simulink model "FlightSim_6DOF"  (R2026b)
settings: Solver=VariableStepAuto
values from neighbouring files (symbols this model uses):
  feet_pos_body_m = [ -1.87  -1.87  -1.87  -1.87 ... (first row only)    [FS_6DOF_config.m]
  g = 9.81    [FS_6DOF_config.m]    (also in hornet_sim_1D_init.m)
  PID_KD_pitch = 0.0    (= 0)    [FS_6DOF_config.m]
  PID_KD_yaw = 0.0    (= 0)    [FS_6DOF_config.m]
  PID_KI_pitch = 0.0    (= 0)    [FS_6DOF_config.m]
  PID_KI_yaw = 0.0    (= 0)    [FS_6DOF_config.m]
  PID_KP_pitch = 0.0    (= 0)    [FS_6DOF_config.m]
  PID_KP_yaw = 0.0    (= 0)    [FS_6DOF_config.m]
  PIDX_KD_pos = 0.0    (= 0)    [FS_6DOF_config.m]
  PIDX_KI_pos = 0.0    (= 0)    [FS_6DOF_config.m]
  PIDX_KP_pos = 0.0    (= 0)    [FS_6DOF_config.m]
  PIDY_KD_pos = 0.0    (= 0)    [FS_6DOF_config.m]
  PIDY_KI_pos = 0.0    (= 0)    [FS_6DOF_config.m]
  PIDY_KP_pos = 0.0    (= 0)    [FS_6DOF_config.m]
  PIDZ_KD_pos = 0.0    (= 0)    [FS_6DOF_config.m]
  PIDZ_KD_vel = 0.0    (= 0)    [FS_6DOF_config.m]
  PIDZ_KI_pos = 0.0    (= 0)    [FS_6DOF_config.m]
  PIDZ_KI_vel = 0.0    (= 0)    [FS_6DOF_config.m]
  PIDZ_KP_pos = 0.0    (= 0)    [FS_6DOF_config.m]
  PIDZ_KP_vel = 0.0    (= 0)    [FS_6DOF_config.m]
  pitch0 = 0.0    (= 0)    [FS_6DOF_config.m]
  Position_Target_inertial = [x_targ; y_targ;z_targ]    [FS_6DOF_config.m]
  roll0 = 0.0    (= 0)    [FS_6DOF_config.m]
  vx0 = 0    [FS_6DOF_config.m]    (also in hornet_sim_1D_init.m)
  vy0 = 0    [FS_6DOF_config.m]
  vz0 = 0    [FS_6DOF_config.m]
  x0 = 0    [FS_6DOF_config.m]    (also in hornet_sim_1D_init.m = 1)
  x_hat_body = [1;0;0]    [FS_6DOF_config.m]
  y0 = 0    [FS_6DOF_config.m]
  yaw0 = 0.0    (= 0)    [FS_6DOF_config.m]
  z0 = 0    [FS_6DOF_config.m]
undefined symbols (not defined in the file or in its folder): DiscIntNeverNeededParam, Lidar_1, Lidar_2, veh, VN300Config
libraries: aerolibutil x8, slpidlib x5, sharedutil x2, matrix_library x1
settings Model: Creator=11and  LastModifiedBy=jet
settings RTWCC: GenCodeOnly=on
settings SimscapeCC: SimscapeLogType=all  SimscapeNominalValues="[{\"value\":\"1\",\"unit\":\"A\"},{\"value\":\"1\",\"unit\":\"bar\"},{\"value\":\"1\",\"unit\":\"cm^2\"},{\"value\":\"1\",\"unit\":\"cm^3/s\"},{\"value\":\"1\",\"unit\":\"kJ/kg\"},{\"value\":\"1\",\"unit\":\"kW\"},{\"value\":\"1\",\"unit\":\"l\"},{\"value\":\"1\",\"unit\":\"N\"},{\"value\":\"1\",\"unit\":\"N*m\"},{\"value\":\"1\",\"unit\":\"V\"},{\"value\":\"0.001\",\"unit\":\"Wb\"}]"  SimscapeUseEnergyAccounting=off

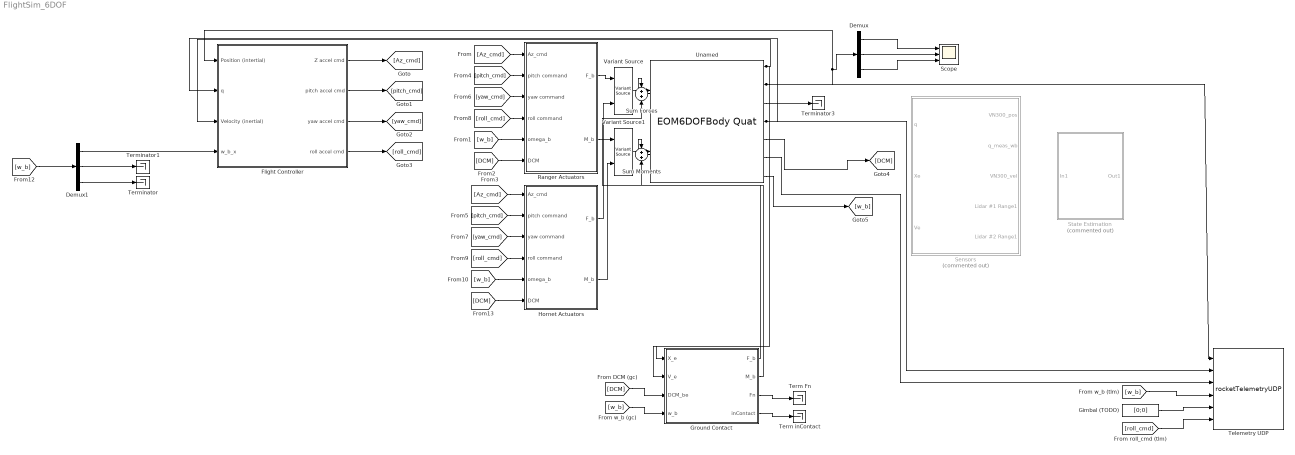
== system FlightSim_6DOF ==
  Demux : Demux  Outputs=3
  Demux1 : Demux  Outputs=3
  Flight Controller : Subsystem
  Gimbal (TODO) : Constant  Value=[0;0]
  Ground Contact : MATLAB Function  TreatAsAtomicUnit=on
  Hornet Actuators : Subsystem
  Ranger Actuators : Subsystem
  Scope : Scope  NumInputPorts=3
      settings: ActiveDisplayYMinimum=-236.81123475820692  ActiveDisplayYMaximum=587.41234905749616
  Sensors : Subsystem  Commented=on
  State Estimation : Subsystem  Commented=on
  Sum Forces : Sum
  Sum Moments : Sum
  Telemetry UDP : M-S-Function  FunctionName=rocketTelemetryUDP
      mask Display:
      | port_label('input', 1, 'position_e');
      | port_label('input', 2, 'quaternion_eb');
      | port_label('input', 3, 'velocity_b');
      | port_label('input', 4, 'omega_b');
      | port_label('input', 5, 'gimbal');
      | port_label('input', 6, 'rcs');
  Term Fn : Terminator
  Term inContact : Terminator
  Terminator : Terminator
  Terminator1 : Terminator
  Terminator3 : Terminator
  Unamed : EOM6DOFBodyQuat  xme_0=[x0 y0 z0]  Vm_0=[vx0 vy0 vz0]  eul_0=[roll0 pitch0 yaw0]  mass_0=veh.m  inertia=veh.I
  Variant Source : VariantSource  VariantControls={VEHICLE == 1, VEHICLE == 2}
  Variant Source1 : VariantSource  VariantControls={VEHICLE == 1, VEHICLE == 2}
  wires:
  Unamed/2 -> Flight Controller/1(Position (intertial)), Demux/1, Telemetry UDP/1, Ground Contact/1(X_e)
  Demux/1 -> Scope/1
  Demux/2 -> Scope/2
  Demux/3 -> Scope/3
  Unamed/4 -> Flight Controller/2(q), Telemetry UDP/2
  Unamed/7 -> [w_b]
  Unamed/1 -> Flight Controller/3(Velocity (inertial)), Ground Contact/2(V_e)
  Demux1/3 -> Terminator/1
  Demux1/2 -> Terminator1/1
  Demux1/1 -> Flight Controller/4(w_b_x)
  Unamed/3 -> Terminator3/1
  Unamed/5 -> [DCM]
  [w_b] -> Demux1/1
  Flight Controller/1(Z accel cmd) -> [Az_cmd]
  Flight Controller/2(pitch accel cmd) -> [pitch_cmd]
  [w_b] -> Hornet Actuators/5(omega_b)
  Ranger Actuators/1(F_b) -> Variant Source/1
  Flight Controller/3(yaw accel cmd) -> [yaw_cmd]
  Flight Controller/4(roll accel cmd) -> [roll_cmd]
  [DCM] -> Hornet Actuators/6(DCM)
  Hornet Actuators/1(F_b) -> Variant Source/2
  Ranger Actuators/2(M_b) -> Variant Source1/1
  Hornet Actuators/2(M_b) -> Variant Source1/2
  [w_b] -> Ranger Actuators/5(omega_b)
  [DCM] -> Ranger Actuators/6(DCM)
  [Az_cmd] -> Ranger Actuators/1(Az_cmd)
  [Az_cmd] -> Hornet Actuators/1(Az_cmd)
  [pitch_cmd] -> Ranger Actuators/2(pitch command)
  [pitch_cmd] -> Hornet Actuators/2(pitch command)
  [yaw_cmd] -> Ranger Actuators/3(yaw command)
  [yaw_cmd] -> Hornet Actuators/3(yaw command)
  [roll_cmd] -> Ranger Actuators/4(roll command)
  [roll_cmd] -> Hornet Actuators/4(roll command)
  Unamed/6 -> Telemetry UDP/3
  [w_b] -> Telemetry UDP/4
  Gimbal (TODO)/1 -> Telemetry UDP/5
  [roll_cmd] -> Telemetry UDP/6
  [DCM] -> Ground Contact/3(DCM_be)
  [w_b] -> Ground Contact/4(w_b)
  Ground Contact/3(Fn) -> Term Fn/1
  Ground Contact/4(inContact) -> Term inContact/1
  Variant Source/1 -> Sum Forces/1
  Ground Contact/1(F_b) -> Sum Forces/2
  Sum Forces/1 -> Unamed/1
  Variant Source1/1 -> Sum Moments/1
  Ground Contact/2(M_b) -> Sum Moments/2
  Sum Moments/1 -> Unamed/2

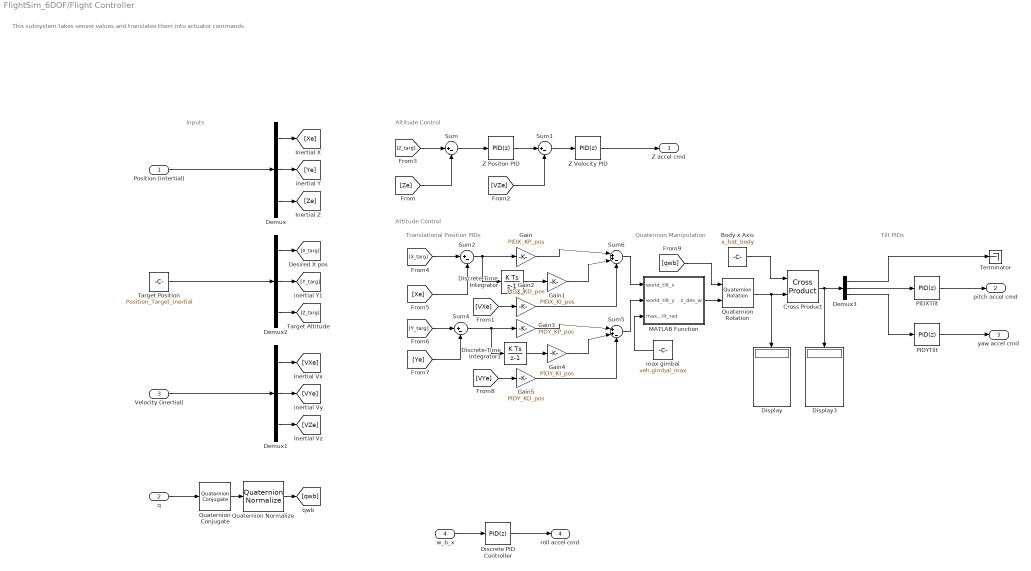
== system FlightSim_6DOF/Flight Controller ==
  note: This subsystem takes sensor values and translates them into actuator commands
  note: Tilt PIDs
  note: Quaternion Manipulation
  note: Translational Position PIDs
  note: Inputs
  note: Attitude Control
  note: Altitude Control
  Position (intertial) : Inport
  q : Inport  Port=2
  Velocity (inertial) : Inport  Port=3
  w_b_x : Inport  Port=4
  Body x Axis : Constant  Value=x_hat_body
  Cross Product : matrix_library/Cross Product
  Demux{,1..3} (4 alike) : Demux  Outputs=3
  Discrete PID Controller : slpidlib/PID Controller  Controller=PID  Form=Parallel  TimeDomain=Discrete-time  UseExternalTs=off  SampleTime=-1  IntegratorMethod=Forward Euler  FilterMethod=Forward Euler  ControllerParametersSource=internal  P=1  I=1  UseKiTs=off  D=0  UseExternalDerivativeSource=off  N=100  UseFilter=on  TunerSelectOption=Transfer Function Based (PID Tuner App)  InitialConditionSource=internal  InitialConditionForIntegrator=0  InitialConditionForFilter=0  DifferentiatorICPrevScaledInput=0  ExternalReset=none  TrackingMode=off  Kt=1  LimitOutput=off  SatLimitsSource=internal  UpperSaturationLimit=inf  LowerSaturationLimit=-inf  LinearizeAsGain=off  AntiWindupMode=none  Kb=1  LimitIntegrator=off  UpperIntegratorSaturationLimit=inf  LowerIntegratorSaturationLimit=-inf  POutMin=[]  POutMax=[]  IOutMin=[]  IOutMax=[]  DOutMin=[]  DOutMax=[]  NOutMin=[]  NOutMax=[]  SumOutMin=[]  SumOutMax=[]  SaturationOutMin=[]  SaturationOutMax=[]  PParamMin=[]  PParamMax=[]  IParamMin=[]  IParamMax=[]  DParamMin=[]  DParamMax=[]  NParamMin=[]  NParamMax=[]  KbParamMin=[]  KbParamMax=[]  KtParamMin=[]  KtParamMax=[]  KbOutMin=[]  KbOutMax=[]  KtOutMin=[]  KtOutMax=[]  IntegratorOutMin=[]  IntegratorOutMax=[]  FilterOutMin=[]  FilterOutMax=[]  SumI1OutMin=[]  SumI1OutMax=[]  SumI2OutMin=[]  SumI2OutMax=[]  SumI3OutMin=[]  SumI3OutMax=[]  SumI4OutMin=[]  SumI4OutMax=[]  SumDOutMin=[]  SumDOutMax=[]  DifferentiatorOutMin=[]  DifferentiatorOutMax=[]  FilterDiffOutCoefMin=[]  FilterDiffOutCoefMax=[]  ReciprocalOutMin=[]  ReciprocalOutMax=[]  SumDenOutMin=[]  SumDenOutMax=[]  SumNumOutMin=[]  SumNumOutMax=[]  DivideOutMin=[]  DivideOutMax=[]  UdiffTsProdOutMin=[]  UdiffTsProdOutMax=[]  NTsProdOutMin=[]  NTsProdOutMax=[]  UintegralTsProdOutMin=[]  UintegralTsProdOutMax=[]  UngainTsProdOutMin=[]  UngainTsProdOutMax=[]  ClampingZeroOutDataTypeStr=Inherit: Inherit via back propagation  ClampingZeroOutMin=[]  ClampingZeroOutMax=[]  FilterDenConstantOutDataTypeStr=Inherit: Inherit via back propagation  FilterDenConstantOutMin=[]  FilterDenConstantOutMax=[]  PCopyOutDataTypeStr=Inherit: Inherit via back propagation  PCopyOutMin=[]  PCopyOutMax=[]  NCopyOutDataTypeStr=Inherit: Inherit via back propagation  NCopyOutMin=[]  NCopyOutMax=[]  IntegratorContinuousStateAttributes=''  IntegratorStateMustResolveToSignalObject=off  IntegratorRTWStateStorageClass=Auto  FilterContinuousStateAttributes=''  FilterStateMustResolveToSignalObject=off  FilterRTWStateStorageClass=Auto  ParallelPVariant=InternalParameters  IdealPVariant=Disabled  IVariant=InternalParameters  DVariant=InternalParameters  IntegratorVariant=Discrete  SatVariant=Disabled  AWVariant=Passthrough  PCopyVariant=Disabled  TRVariant=Disabled  FdbkBlocksVariant=Forward  IdealPFdbkVariant=Disabled  SatFdbkVariant=Disabled  DerivativeFilterVariant=ForwardEulerFilter  NVariant=InternalParameters  NCopyVariant=Disabled  FilterICVariant=InternalICsFilter  IntegratorICVariant=InternalICs  ExternalResetVariant=Disabled  TRSumVariant=Passthrough  SumFdbkVariant=Disabled  SumVariant=Sum_PID  TsampFilterVariant=InternalTs  TsampNgainVariant=Passthrough  TsampIntegralVariant=Disabled_SignalSpec  ExternalSaturationOutDataTypeStr=Inherit: Same as second input  DerivativeSourceVariant=ErrorSignal  PreIntVariant=InternalPreInt
      settings: LibrarySourceBlock=simulink/Discrete/Discrete PID Controller
  Discrete-Time Integrator : DiscreteIntegrator  SampleTime=-1  ICPrevOutput=DiscIntNeverNeededParam  ICPrevScaledInput=DiscIntNeverNeededParam
  Discrete-Time Integrator1 : DiscreteIntegrator  SampleTime=-1  ICPrevOutput=DiscIntNeverNeededParam  ICPrevScaledInput=DiscIntNeverNeededParam
  Display : Display
  Display3 : Display
  Gain : Gain  Gain=PIDX_KP_pos
  Gain1 : Gain  Gain=PIDX_KI_pos
  Gain2 : Gain  Gain=PIDX_KD_pos
  Gain3 : Gain  Gain=PIDY_KP_pos
  Gain4 : Gain  Gain=PIDY_KI_pos
  Gain5 : Gain  Gain=PIDY_KD_pos
  MATLAB Function : MATLAB Function  TreatAsAtomicUnit=on
  PIDXTilt : slpidlib/PID Controller  Controller=PID  Form=Parallel  TimeDomain=Discrete-time  UseExternalTs=off  SampleTime=-1  IntegratorMethod=Forward Euler  FilterMethod=Forward Euler  ControllerParametersSource=internal  P=PID_KP_pitch  I=PID_KI_pitch  UseKiTs=off  D=PID_KD_pitch  UseExternalDerivativeSource=off  N=100  UseFilter=on  TunerSelectOption=Transfer Function Based (PID Tuner App)  InitialConditionSource=internal  InitialConditionForIntegrator=0  InitialConditionForFilter=0  DifferentiatorICPrevScaledInput=0  ExternalReset=none  TrackingMode=off  Kt=1  LimitOutput=off  SatLimitsSource=internal  UpperSaturationLimit=inf  LowerSaturationLimit=-inf  LinearizeAsGain=off  AntiWindupMode=none  Kb=1  LimitIntegrator=off  UpperIntegratorSaturationLimit=inf  LowerIntegratorSaturationLimit=-inf  POutMin=[]  POutMax=[]  IOutMin=[]  IOutMax=[]  DOutMin=[]  DOutMax=[]  NOutMin=[]  NOutMax=[]  SumOutMin=[]  SumOutMax=[]  SaturationOutMin=[]  SaturationOutMax=[]  PParamMin=[]  PParamMax=[]  IParamMin=[]  IParamMax=[]  DParamMin=[]  DParamMax=[]  NParamMin=[]  NParamMax=[]  KbParamMin=[]  KbParamMax=[]  KtParamMin=[]  KtParamMax=[]  KbOutMin=[]  KbOutMax=[]  KtOutMin=[]  KtOutMax=[]  IntegratorOutMin=[]  IntegratorOutMax=[]  FilterOutMin=[]  FilterOutMax=[]  SumI1OutMin=[]  SumI1OutMax=[]  SumI2OutMin=[]  SumI2OutMax=[]  SumI3OutMin=[]  SumI3OutMax=[]  SumI4OutMin=[]  SumI4OutMax=[]  SumDOutMin=[]  SumDOutMax=[]  DifferentiatorOutMin=[]  DifferentiatorOutMax=[]  FilterDiffOutCoefMin=[]  FilterDiffOutCoefMax=[]  ReciprocalOutMin=[]  ReciprocalOutMax=[]  SumDenOutMin=[]  SumDenOutMax=[]  SumNumOutMin=[]  SumNumOutMax=[]  DivideOutMin=[]  DivideOutMax=[]  UdiffTsProdOutMin=[]  UdiffTsProdOutMax=[]  NTsProdOutMin=[]  NTsProdOutMax=[]  UintegralTsProdOutMin=[]  UintegralTsProdOutMax=[]  UngainTsProdOutMin=[]  UngainTsProdOutMax=[]  ClampingZeroOutDataTypeStr=Inherit: Inherit via back propagation  ClampingZeroOutMin=[]  ClampingZeroOutMax=[]  FilterDenConstantOutDataTypeStr=Inherit: Inherit via back propagation  FilterDenConstantOutMin=[]  FilterDenConstantOutMax=[]  PCopyOutDataTypeStr=Inherit: Inherit via back propagation  PCopyOutMin=[]  PCopyOutMax=[]  NCopyOutDataTypeStr=Inherit: Inherit via back propagation  NCopyOutMin=[]  NCopyOutMax=[]  IntegratorContinuousStateAttributes=''  IntegratorStateMustResolveToSignalObject=off  IntegratorRTWStateStorageClass=Auto  FilterContinuousStateAttributes=''  FilterStateMustResolveToSignalObject=off  FilterRTWStateStorageClass=Auto  ParallelPVariant=InternalParameters  IdealPVariant=Disabled  IVariant=InternalParameters  DVariant=InternalParameters  IntegratorVariant=Discrete  SatVariant=Disabled  AWVariant=Passthrough  PCopyVariant=Disabled  TRVariant=Disabled  FdbkBlocksVariant=Forward  IdealPFdbkVariant=Disabled  SatFdbkVariant=Disabled  DerivativeFilterVariant=ForwardEulerFilter  NVariant=InternalParameters  NCopyVariant=Disabled  FilterICVariant=InternalICsFilter  IntegratorICVariant=InternalICs  ExternalResetVariant=Disabled  TRSumVariant=Passthrough  SumFdbkVariant=Disabled  SumVariant=Sum_PID  TsampFilterVariant=InternalTs  TsampNgainVariant=Passthrough  TsampIntegralVariant=Disabled_SignalSpec  ExternalSaturationOutDataTypeStr=Inherit: Same as second input  DerivativeSourceVariant=ErrorSignal  PreIntVariant=InternalPreInt
      settings: LibrarySourceBlock=simulink/Discrete/Discrete PID Controller
  PIDYTilt : slpidlib/PID Controller  Controller=PID  Form=Parallel  TimeDomain=Discrete-time  UseExternalTs=off  SampleTime=-1  IntegratorMethod=Forward Euler  FilterMethod=Forward Euler  ControllerParametersSource=internal  P=PID_KP_yaw  I=PID_KI_yaw  UseKiTs=off  D=PID_KD_yaw  UseExternalDerivativeSource=off  N=100  UseFilter=on  TunerSelectOption=Transfer Function Based (PID Tuner App)  InitialConditionSource=internal  InitialConditionForIntegrator=0  InitialConditionForFilter=0  DifferentiatorICPrevScaledInput=0  ExternalReset=none  TrackingMode=off  Kt=1  LimitOutput=off  SatLimitsSource=internal  UpperSaturationLimit=inf  LowerSaturationLimit=-inf  LinearizeAsGain=off  AntiWindupMode=none  Kb=1  LimitIntegrator=off  UpperIntegratorSaturationLimit=inf  LowerIntegratorSaturationLimit=-inf  POutMin=[]  POutMax=[]  IOutMin=[]  IOutMax=[]  DOutMin=[]  DOutMax=[]  NOutMin=[]  NOutMax=[]  SumOutMin=[]  SumOutMax=[]  SaturationOutMin=[]  SaturationOutMax=[]  PParamMin=[]  PParamMax=[]  IParamMin=[]  IParamMax=[]  DParamMin=[]  DParamMax=[]  NParamMin=[]  NParamMax=[]  KbParamMin=[]  KbParamMax=[]  KtParamMin=[]  KtParamMax=[]  KbOutMin=[]  KbOutMax=[]  KtOutMin=[]  KtOutMax=[]  IntegratorOutMin=[]  IntegratorOutMax=[]  FilterOutMin=[]  FilterOutMax=[]  SumI1OutMin=[]  SumI1OutMax=[]  SumI2OutMin=[]  SumI2OutMax=[]  SumI3OutMin=[]  SumI3OutMax=[]  SumI4OutMin=[]  SumI4OutMax=[]  SumDOutMin=[]  SumDOutMax=[]  DifferentiatorOutMin=[]  DifferentiatorOutMax=[]  FilterDiffOutCoefMin=[]  FilterDiffOutCoefMax=[]  ReciprocalOutMin=[]  ReciprocalOutMax=[]  SumDenOutMin=[]  SumDenOutMax=[]  SumNumOutMin=[]  SumNumOutMax=[]  DivideOutMin=[]  DivideOutMax=[]  UdiffTsProdOutMin=[]  UdiffTsProdOutMax=[]  NTsProdOutMin=[]  NTsProdOutMax=[]  UintegralTsProdOutMin=[]  UintegralTsProdOutMax=[]  UngainTsProdOutMin=[]  UngainTsProdOutMax=[]  ClampingZeroOutDataTypeStr=Inherit: Inherit via back propagation  ClampingZeroOutMin=[]  ClampingZeroOutMax=[]  FilterDenConstantOutDataTypeStr=Inherit: Inherit via back propagation  FilterDenConstantOutMin=[]  FilterDenConstantOutMax=[]  PCopyOutDataTypeStr=Inherit: Inherit via back propagation  PCopyOutMin=[]  PCopyOutMax=[]  NCopyOutDataTypeStr=Inherit: Inherit via back propagation  NCopyOutMin=[]  NCopyOutMax=[]  IntegratorContinuousStateAttributes=''  IntegratorStateMustResolveToSignalObject=off  IntegratorRTWStateStorageClass=Auto  FilterContinuousStateAttributes=''  FilterStateMustResolveToSignalObject=off  FilterRTWStateStorageClass=Auto  ParallelPVariant=InternalParameters  IdealPVariant=Disabled  IVariant=InternalParameters  DVariant=InternalParameters  IntegratorVariant=Discrete  SatVariant=Disabled  AWVariant=Passthrough  PCopyVariant=Disabled  TRVariant=Disabled  FdbkBlocksVariant=Forward  IdealPFdbkVariant=Disabled  SatFdbkVariant=Disabled  DerivativeFilterVariant=ForwardEulerFilter  NVariant=InternalParameters  NCopyVariant=Disabled  FilterICVariant=InternalICsFilter  IntegratorICVariant=InternalICs  ExternalResetVariant=Disabled  TRSumVariant=Passthrough  SumFdbkVariant=Disabled  SumVariant=Sum_PID  TsampFilterVariant=InternalTs  TsampNgainVariant=Passthrough  TsampIntegralVariant=Disabled_SignalSpec  ExternalSaturationOutDataTypeStr=Inherit: Same as second input  DerivativeSourceVariant=ErrorSignal  PreIntVariant=InternalPreInt
      settings: LibrarySourceBlock=simulink/Discrete/Discrete PID Controller
  Quaternion Conjugate : aerolibutil/Quaternion Conjugate
  Quaternion Normalize : sharedutil/Quaternion Normalize  aMode=aMode
  Quaternion Rotation : aerolibutil/Quaternion Rotation
  Sum{,1..2,4} (4 alike) : Sum  Inputs=|+-
  Sum5 : Sum  Inputs=|++-
  Sum6 : Sum  Inputs=|++-
  Target Position : Constant  Value=Position_Target_inertial
  Terminator : Terminator
  Z Positon PID : slpidlib/PID Controller  Controller=PID  Form=Parallel  TimeDomain=Discrete-time  UseExternalTs=off  SampleTime=-1  IntegratorMethod=Forward Euler  FilterMethod=Forward Euler  ControllerParametersSource=internal  P=PIDZ_KP_pos  I=PIDZ_KI_pos  UseKiTs=off  D=PIDZ_KD_pos  UseExternalDerivativeSource=off  N=100  UseFilter=on  TunerSelectOption=Transfer Function Based (PID Tuner App)  InitialConditionSource=internal  InitialConditionForIntegrator=0  InitialConditionForFilter=0  DifferentiatorICPrevScaledInput=0  ExternalReset=none  TrackingMode=off  Kt=1  LimitOutput=off  SatLimitsSource=internal  UpperSaturationLimit=inf  LowerSaturationLimit=-inf  LinearizeAsGain=off  AntiWindupMode=none  Kb=1  LimitIntegrator=off  UpperIntegratorSaturationLimit=inf  LowerIntegratorSaturationLimit=-inf  POutMin=[]  POutMax=[]  IOutMin=[]  IOutMax=[]  DOutMin=[]  DOutMax=[]  NOutMin=[]  NOutMax=[]  SumOutMin=[]  SumOutMax=[]  SaturationOutMin=[]  SaturationOutMax=[]  PParamMin=[]  PParamMax=[]  IParamMin=[]  IParamMax=[]  DParamMin=[]  DParamMax=[]  NParamMin=[]  NParamMax=[]  KbParamMin=[]  KbParamMax=[]  KtParamMin=[]  KtParamMax=[]  KbOutMin=[]  KbOutMax=[]  KtOutMin=[]  KtOutMax=[]  IntegratorOutMin=[]  IntegratorOutMax=[]  FilterOutMin=[]  FilterOutMax=[]  SumI1OutMin=[]  SumI1OutMax=[]  SumI2OutMin=[]  SumI2OutMax=[]  SumI3OutMin=[]  SumI3OutMax=[]  SumI4OutMin=[]  SumI4OutMax=[]  SumDOutMin=[]  SumDOutMax=[]  DifferentiatorOutMin=[]  DifferentiatorOutMax=[]  FilterDiffOutCoefMin=[]  FilterDiffOutCoefMax=[]  ReciprocalOutMin=[]  ReciprocalOutMax=[]  SumDenOutMin=[]  SumDenOutMax=[]  SumNumOutMin=[]  SumNumOutMax=[]  DivideOutMin=[]  DivideOutMax=[]  UdiffTsProdOutMin=[]  UdiffTsProdOutMax=[]  NTsProdOutMin=[]  NTsProdOutMax=[]  UintegralTsProdOutMin=[]  UintegralTsProdOutMax=[]  UngainTsProdOutMin=[]  UngainTsProdOutMax=[]  ClampingZeroOutDataTypeStr=Inherit: Inherit via back propagation  ClampingZeroOutMin=[]  ClampingZeroOutMax=[]  FilterDenConstantOutDataTypeStr=Inherit: Inherit via back propagation  FilterDenConstantOutMin=[]  FilterDenConstantOutMax=[]  PCopyOutDataTypeStr=Inherit: Inherit via back propagation  PCopyOutMin=[]  PCopyOutMax=[]  NCopyOutDataTypeStr=Inherit: Inherit via back propagation  NCopyOutMin=[]  NCopyOutMax=[]  IntegratorContinuousStateAttributes=''  IntegratorStateMustResolveToSignalObject=off  IntegratorRTWStateStorageClass=Auto  FilterContinuousStateAttributes=''  FilterStateMustResolveToSignalObject=off  FilterRTWStateStorageClass=Auto  ParallelPVariant=InternalParameters  IdealPVariant=Disabled  IVariant=InternalParameters  DVariant=InternalParameters  IntegratorVariant=Discrete  SatVariant=Disabled  AWVariant=Passthrough  PCopyVariant=Disabled  TRVariant=Disabled  FdbkBlocksVariant=Forward  IdealPFdbkVariant=Disabled  SatFdbkVariant=Disabled  DerivativeFilterVariant=ForwardEulerFilter  NVariant=InternalParameters  NCopyVariant=Disabled  FilterICVariant=InternalICsFilter  IntegratorICVariant=InternalICs  ExternalResetVariant=Disabled  TRSumVariant=Passthrough  SumFdbkVariant=Disabled  SumVariant=Sum_PID  TsampFilterVariant=InternalTs  TsampNgainVariant=Passthrough  TsampIntegralVariant=Disabled_SignalSpec  ExternalSaturationOutDataTypeStr=Inherit: Same as second input  DerivativeSourceVariant=ErrorSignal  PreIntVariant=InternalPreInt
      settings: LibrarySourceBlock=simulink/Discrete/Discrete PID Controller
  Z Velocity PID : slpidlib/PID Controller  Controller=PID  Form=Parallel  TimeDomain=Discrete-time  UseExternalTs=off  SampleTime=-1  IntegratorMethod=Forward Euler  FilterMethod=Forward Euler  ControllerParametersSource=internal  P=PIDZ_KP_vel  I=PIDZ_KI_vel  UseKiTs=off  D=PIDZ_KD_vel  UseExternalDerivativeSource=off  N=100  UseFilter=on  TunerSelectOption=Transfer Function Based (PID Tuner App)  InitialConditionSource=internal  InitialConditionForIntegrator=0  InitialConditionForFilter=0  DifferentiatorICPrevScaledInput=0  ExternalReset=none  TrackingMode=off  Kt=1  LimitOutput=off  SatLimitsSource=internal  UpperSaturationLimit=inf  LowerSaturationLimit=-inf  LinearizeAsGain=off  AntiWindupMode=none  Kb=1  LimitIntegrator=off  UpperIntegratorSaturationLimit=inf  LowerIntegratorSaturationLimit=-inf  POutMin=[]  POutMax=[]  IOutMin=[]  IOutMax=[]  DOutMin=[]  DOutMax=[]  NOutMin=[]  NOutMax=[]  SumOutMin=[]  SumOutMax=[]  SaturationOutMin=[]  SaturationOutMax=[]  PParamMin=[]  PParamMax=[]  IParamMin=[]  IParamMax=[]  DParamMin=[]  DParamMax=[]  NParamMin=[]  NParamMax=[]  KbParamMin=[]  KbParamMax=[]  KtParamMin=[]  KtParamMax=[]  KbOutMin=[]  KbOutMax=[]  KtOutMin=[]  KtOutMax=[]  IntegratorOutMin=[]  IntegratorOutMax=[]  FilterOutMin=[]  FilterOutMax=[]  SumI1OutMin=[]  SumI1OutMax=[]  SumI2OutMin=[]  SumI2OutMax=[]  SumI3OutMin=[]  SumI3OutMax=[]  SumI4OutMin=[]  SumI4OutMax=[]  SumDOutMin=[]  SumDOutMax=[]  DifferentiatorOutMin=[]  DifferentiatorOutMax=[]  FilterDiffOutCoefMin=[]  FilterDiffOutCoefMax=[]  ReciprocalOutMin=[]  ReciprocalOutMax=[]  SumDenOutMin=[]  SumDenOutMax=[]  SumNumOutMin=[]  SumNumOutMax=[]  DivideOutMin=[]  DivideOutMax=[]  UdiffTsProdOutMin=[]  UdiffTsProdOutMax=[]  NTsProdOutMin=[]  NTsProdOutMax=[]  UintegralTsProdOutMin=[]  UintegralTsProdOutMax=[]  UngainTsProdOutMin=[]  UngainTsProdOutMax=[]  ClampingZeroOutDataTypeStr=Inherit: Inherit via back propagation  ClampingZeroOutMin=[]  ClampingZeroOutMax=[]  FilterDenConstantOutDataTypeStr=Inherit: Inherit via back propagation  FilterDenConstantOutMin=[]  FilterDenConstantOutMax=[]  PCopyOutDataTypeStr=Inherit: Inherit via back propagation  PCopyOutMin=[]  PCopyOutMax=[]  NCopyOutDataTypeStr=Inherit: Inherit via back propagation  NCopyOutMin=[]  NCopyOutMax=[]  IntegratorContinuousStateAttributes=''  IntegratorStateMustResolveToSignalObject=off  IntegratorRTWStateStorageClass=Auto  FilterContinuousStateAttributes=''  FilterStateMustResolveToSignalObject=off  FilterRTWStateStorageClass=Auto  ParallelPVariant=InternalParameters  IdealPVariant=Disabled  IVariant=InternalParameters  DVariant=InternalParameters  IntegratorVariant=Discrete  SatVariant=Disabled  AWVariant=Passthrough  PCopyVariant=Disabled  TRVariant=Disabled  FdbkBlocksVariant=Forward  IdealPFdbkVariant=Disabled  SatFdbkVariant=Disabled  DerivativeFilterVariant=ForwardEulerFilter  NVariant=InternalParameters  NCopyVariant=Disabled  FilterICVariant=InternalICsFilter  IntegratorICVariant=InternalICs  ExternalResetVariant=Disabled  TRSumVariant=Passthrough  SumFdbkVariant=Disabled  SumVariant=Sum_PID  TsampFilterVariant=InternalTs  TsampNgainVariant=Passthrough  TsampIntegralVariant=Disabled_SignalSpec  ExternalSaturationOutDataTypeStr=Inherit: Same as second input  DerivativeSourceVariant=ErrorSignal  PreIntVariant=InternalPreInt
      settings: LibrarySourceBlock=simulink/Discrete/Discrete PID Controller
  max gimbal : Constant  Value=veh.gimbal_max
  Z accel cmd : Outport
  pitch accel cmd : Outport  Port=2
  yaw accel cmd : Outport  Port=3
  roll accel cmd : Outport  Port=4
  wires:
  [Z_targ] -> Sum/1
  Sum/1 -> Z Positon PID/1
  Z Velocity PID/1 -> Z accel cmd/1
  Position (intertial)/1 -> Demux/1
  Demux/1 -> [Xe]
  [Ze] -> Sum/2
  Z Positon PID/1 -> Sum1/1
  Demux1/1 -> [VXe]
  Demux1/2 -> [VYe]
  Demux1/3 -> [VZe]
  [VZe] -> Sum1/2
  Sum1/1 -> Z Velocity PID/1
  Demux2/1 -> [X_targ]
  Demux2/2 -> [Y_targ]
  Demux2/3 -> [Z_targ]
  Sum2/1 -> Discrete-Time Integrator/1, Gain/1
  [X_targ] -> Sum2/1
  [Xe] -> Sum2/2
  [Y_targ] -> Sum4/1
  [Ye] -> Sum4/2
  [VXe] -> Gain2/1
  Gain/1 -> Sum6/1
  Gain2/1 -> Sum6/3
  PIDXTilt/1 -> pitch accel cmd/1
  PIDYTilt/1 -> yaw accel cmd/1
  Gain5/1 -> Sum5/3
  [VYe] -> Gain5/1
  Sum4/1 -> Discrete-Time Integrator1/1, Gain3/1
  Gain3/1 -> Sum5/1
  Sum6/1 -> MATLAB Function/1(world_tilt_x)
  Sum5/1 -> MATLAB Function/2(world_tilt_y)
  MATLAB Function/1(z_des_w) -> Quaternion Rotation/2
  Quaternion Rotation/1 -> Cross Product/2, Display/1
  Body x Axis/1 -> Cross Product/1
  Cross Product/1 -> Demux3/1, Display3/1
  [qwb] -> Quaternion Rotation/1
  Demux3/2 -> PIDXTilt/1
  Demux3/1 -> Terminator/1
  Demux3/3 -> PIDYTilt/1
  Demux/2 -> [Ye]
  Demux/3 -> [Ze]
  Target Position/1 -> Demux2/1
  Quaternion Conjugate/1 -> Quaternion Normalize/1
  q/1 -> Quaternion Conjugate/1
  Quaternion Normalize/1 -> [qwb]
  max gimbal/1 -> MATLAB Function/3(max_tilt_rad)
  Discrete-Time Integrator1/1 -> Gain4/1
  Gain4/1 -> Sum5/2
  Discrete-Time Integrator/1 -> Gain1/1
  Gain1/1 -> Sum6/2
  Velocity (inertial)/1 -> Demux1/1
  w_b_x/1 -> Discrete PID Controller/1
  Discrete PID Controller/1 -> roll accel cmd/1

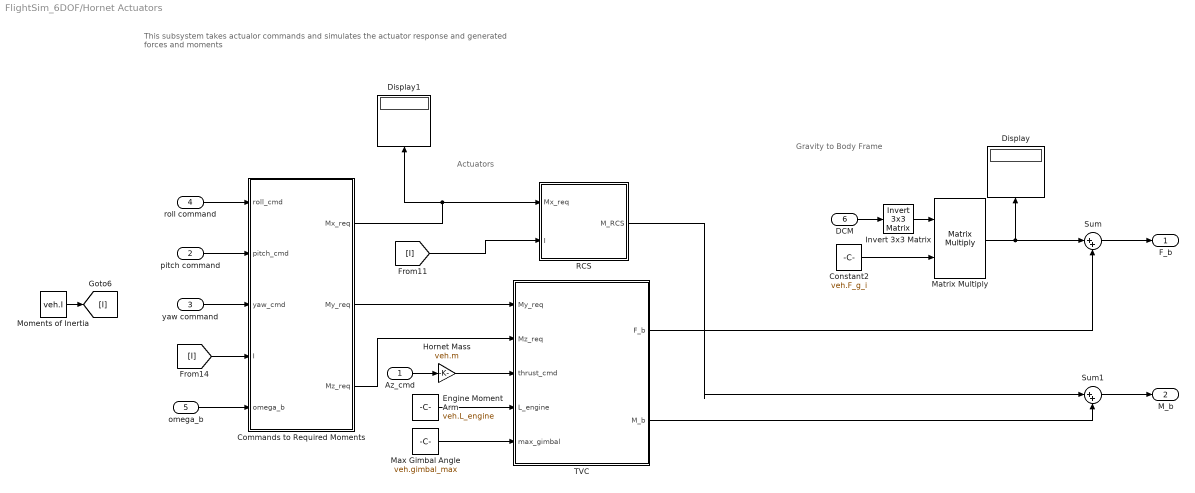
== system FlightSim_6DOF/Hornet Actuators ==
  note: This subsystem takes actualor commands and simulates the actuator response and generated forces and moments
  note: Actuators
  note: Gravity to Body Frame
  Az_cmd : Inport
  pitch command : Inport  Port=2
  yaw command : Inport  Port=3
  roll command : Inport  Port=4
  omega_b : Inport  Port=5
  DCM : Inport  Port=6
  Commands to Required Moments : MATLAB Function  TreatAsAtomicUnit=on
  Constant2 : Constant  Value=veh.F_g_i
  Display : Display
  Display1 : Display
  Engine Moment Arm : Constant  Value=veh.L_engine
  Hornet Mass : Gain  Gain=veh.m
  Invert 3x3 Matrix : aerolibutil/Invert  3x3 Matrix
  Matrix Multiply : Product  Multiplication=Matrix(*)
  Max Gimbal Angle : Constant  Value=veh.gimbal_max
  Moments of Inertia : Constant  Value=veh.I
  RCS : MATLAB Function  TreatAsAtomicUnit=on
  Sum : Sum  Inputs=|++
  Sum1 : Sum  Inputs=|++
  TVC : MATLAB Function  TreatAsAtomicUnit=on
  F_b : Outport
  M_b : Outport  Port=2
  wires:
  RCS/1(M_RCS) -> Sum1/1
  Matrix Multiply/1 -> Sum/1, Display/1
  roll command/1 -> Commands to Required Moments/1(roll_cmd)
  Commands to Required Moments/1(Mx_req) -> RCS/1(Mx_req), Display1/1
  Engine Moment Arm/1 -> TVC/4(L_engine)
  DCM/1 -> Invert 3x3 Matrix/1
  Moments of Inertia/1 -> [I]
  Invert 3x3 Matrix/1 -> Matrix Multiply/1
  Sum/1 -> F_b/1
  pitch command/1 -> Commands to Required Moments/2(pitch_cmd)
  [I] -> RCS/2(I)
  Constant2/1 -> Matrix Multiply/2
  yaw command/1 -> Commands to Required Moments/3(yaw_cmd)
  Commands to Required Moments/3(Mz_req) -> TVC/2(Mz_req)
  Commands to Required Moments/2(My_req) -> TVC/1(My_req)
  TVC/1(F_b) -> Sum/2
  [I] -> Commands to Required Moments/4(I)
  Az_cmd/1 -> Hornet Mass/1
  Hornet Mass/1 -> TVC/3(thrust_cmd)
  Sum1/1 -> M_b/1
  omega_b/1 -> Commands to Required Moments/5(omega_b)
  TVC/2(M_b) -> Sum1/2
  Max Gimbal Angle/1 -> TVC/5(max_gimbal)

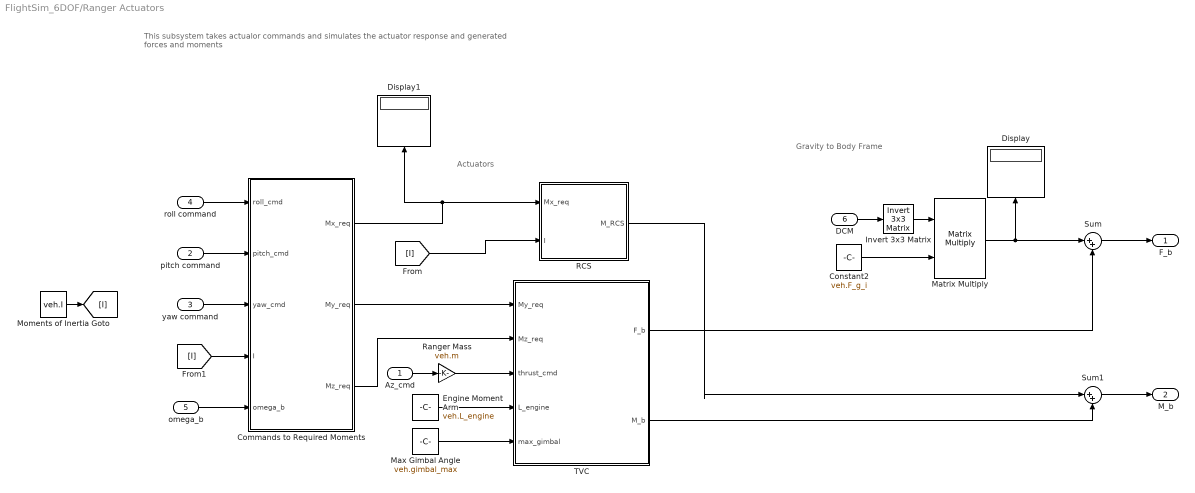
== system FlightSim_6DOF/Ranger Actuators ==
  note: This subsystem takes actualor commands and simulates the actuator response and generated forces and moments
  note: Actuators
  note: Gravity to Body Frame
  Az_cmd : Inport
  pitch command : Inport  Port=2
  yaw command : Inport  Port=3
  roll command : Inport  Port=4
  omega_b : Inport  Port=5
  DCM : Inport  Port=6
  Commands to Required Moments : MATLAB Function  TreatAsAtomicUnit=on
  Constant2 : Constant  Value=veh.F_g_i
  Display : Display
  Display1 : Display
  Engine Moment Arm : Constant  Value=veh.L_engine
  Invert 3x3 Matrix : aerolibutil/Invert  3x3 Matrix
  Matrix Multiply : Product  Multiplication=Matrix(*)
  Max Gimbal Angle : Constant  Value=veh.gimbal_max
  Moments of Inertia : Constant  Value=veh.I
  RCS : MATLAB Function  TreatAsAtomicUnit=on
  Ranger Mass : Gain  Gain=veh.m
  Sum : Sum  Inputs=|++
  Sum1 : Sum  Inputs=|++
  TVC : MATLAB Function  TreatAsAtomicUnit=on
  F_b : Outport
  M_b : Outport  Port=2
  wires:
  DCM/1 -> Invert 3x3 Matrix/1
  roll command/1 -> Commands to Required Moments/1(roll_cmd)
  RCS/1(M_RCS) -> Sum1/1
  Commands to Required Moments/1(Mx_req) -> RCS/1(Mx_req), Display1/1
  Invert 3x3 Matrix/1 -> Matrix Multiply/1
  Matrix Multiply/1 -> Sum/1, Display/1
  Ranger Mass/1 -> TVC/3(thrust_cmd)
  Sum/1 -> F_b/1
  pitch command/1 -> Commands to Required Moments/2(pitch_cmd)
  Az_cmd/1 -> Ranger Mass/1
  [I] -> RCS/2(I)
  Constant2/1 -> Matrix Multiply/2
  Moments of Inertia/1 -> [I]
  yaw command/1 -> Commands to Required Moments/3(yaw_cmd)
  Engine Moment Arm/1 -> TVC/4(L_engine)
  Commands to Required Moments/2(My_req) -> TVC/1(My_req)
  TVC/1(F_b) -> Sum/2
  [I] -> Commands to Required Moments/4(I)
  Commands to Required Moments/3(Mz_req) -> TVC/2(Mz_req)
  Sum1/1 -> M_b/1
  omega_b/1 -> Commands to Required Moments/5(omega_b)
  TVC/2(M_b) -> Sum1/2
  Max Gimbal Angle/1 -> TVC/5(max_gimbal)

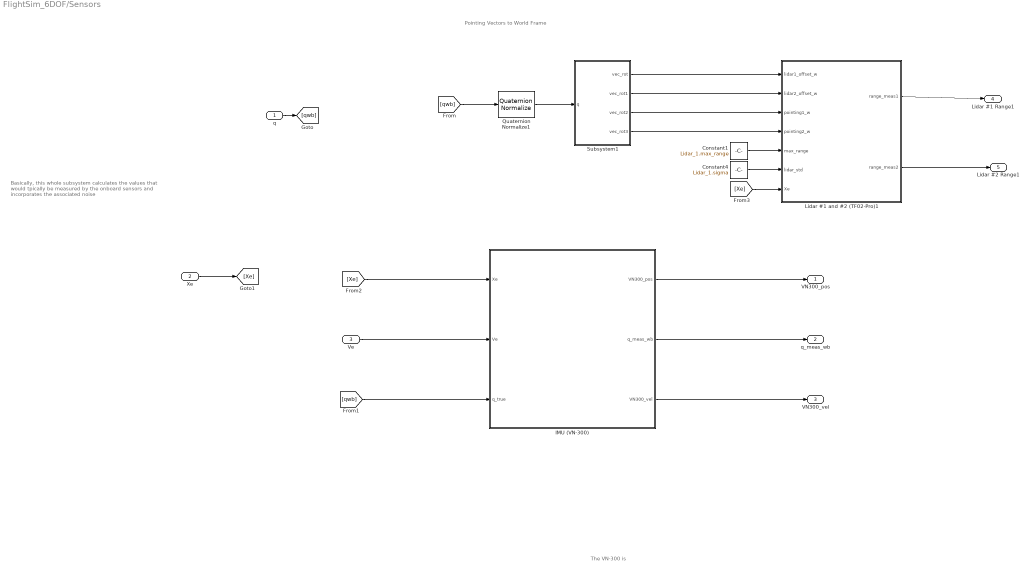
== system FlightSim_6DOF/Sensors ==
  note: The VN-300 is
  note: Basically, this whole subsystem calculates the values that would tpically be measured by the onboard sensors and incorporates the associated noise
  note: Pointing Vectors to World Frame
  q : Inport
  Xe : Inport  Port=2
  Ve : Inport  Port=3
  Constant1 : Constant  Value=Lidar_1.max_range
  Constant4 : Constant  Value=Lidar_1.sigma
  IMU (VN-300) : Subsystem
  Lidar #1 and #2 (TF02-Pro)1 : MATLAB Function  TreatAsAtomicUnit=on  SystemSampleTime=1/Lidar_1.sample_rate
  Quaternion Normalize1 : sharedutil/Quaternion Normalize  aMode=aMode
  Subsystem1 : Subsystem
  VN300_pos : Outport
  q_meas_wb : Outport  Port=2
  VN300_vel : Outport  Port=3
  Lidar #1 Range1 : Outport  Port=4
  Lidar #2 Range1 : Outport  Port=5
  wires:
  Ve/1 -> IMU (VN-300)/2(Ve)
  IMU (VN-300)/1(VN300_pos) -> VN300_pos/1
  IMU (VN-300)/2(q_meas_wb) -> q_meas_wb/1
  IMU (VN-300)/3(VN300_vel) -> VN300_vel/1
  q/1 -> [qwb]
  [qwb] -> IMU (VN-300)/3(q_true)
  Lidar #1 and #2 (TF02-Pro)1/1(range_meas1) -> Lidar #1 Range1/1
  Subsystem1/2(vec_rot1) -> Lidar #1 and #2 (TF02-Pro)1/2(lidar2_offset_w)
  Subsystem1/3(vec_rot2) -> Lidar #1 and #2 (TF02-Pro)1/3(pointing1_w)
  Constant1/1 -> Lidar #1 and #2 (TF02-Pro)1/5(max_range)
  Lidar #1 and #2 (TF02-Pro)1/2(range_meas2) -> Lidar #2 Range1/1
  Subsystem1/4(vec_rot3) -> Lidar #1 and #2 (TF02-Pro)1/4(pointing2_w)
  [Xe] -> Lidar #1 and #2 (TF02-Pro)1/7(Xe)
  Constant4/1 -> Lidar #1 and #2 (TF02-Pro)1/6(lidar_std)
  Quaternion Normalize1/1 -> Subsystem1/1(q)
  Subsystem1/1(vec_rot) -> Lidar #1 and #2 (TF02-Pro)1/1(lidar1_offset_w)
  [qwb] -> Quaternion Normalize1/1
  Xe/1 -> [Xe]
  [Xe] -> IMU (VN-300)/1(Xe)

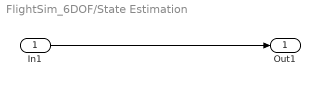
== system FlightSim_6DOF/State Estimation ==
  In1 : Inport
  Out1 : Outport
  wires:
  In1/1 -> Out1/1

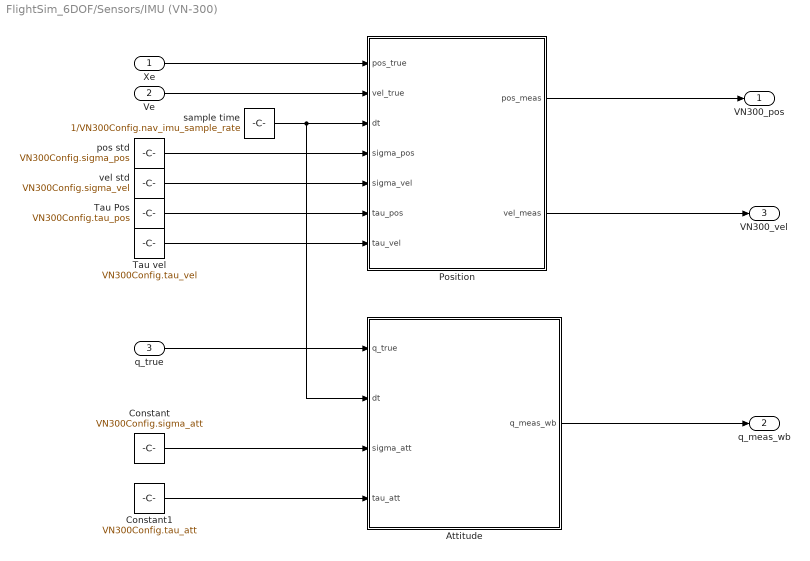
== system FlightSim_6DOF/Sensors/IMU (VN-300) ==
  Xe : Inport
  Ve : Inport  Port=2
  q_true : Inport  Port=3
  Attitude : MATLAB Function  TreatAsAtomicUnit=on  SystemSampleTime=1/VN300Config.nav_imu_sample_rate
  Constant : Constant  Value=VN300Config.sigma_att
  Constant1 : Constant  Value=VN300Config.tau_att
  Position : MATLAB Function  TreatAsAtomicUnit=on  SystemSampleTime=1/VN300Config.nav_imu_sample_rate
  Tau Pos : Constant  Value=VN300Config.tau_pos
  Tau vel : Constant  Value=VN300Config.tau_vel
  pos std : Constant  Value=VN300Config.sigma_pos
  sample time : Constant  Value=1/VN300Config.nav_imu_sample_rate
  vel std : Constant  Value=VN300Config.sigma_vel
  VN300_pos : Outport
  q_meas_wb : Outport  Port=2
  VN300_vel : Outport  Port=3
  wires:
  sample time/1 -> Attitude/2(dt), Position/3(dt)
  Xe/1 -> Position/1(pos_true)
  Ve/1 -> Position/2(vel_true)
  pos std/1 -> Position/4(sigma_pos)
  vel std/1 -> Position/5(sigma_vel)
  Tau Pos/1 -> Position/6(tau_pos)
  Tau vel/1 -> Position/7(tau_vel)
  q_true/1 -> Attitude/1(q_true)
  Attitude/1(q_meas_wb) -> q_meas_wb/1
  Constant/1 -> Attitude/3(sigma_att)
  Constant1/1 -> Attitude/4(tau_att)
  Position/1(pos_meas) -> VN300_pos/1
  Position/2(vel_meas) -> VN300_vel/1

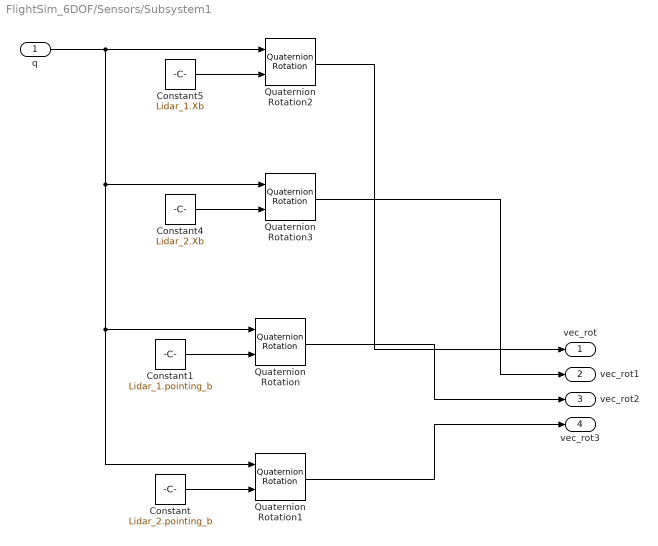
== system FlightSim_6DOF/Sensors/Subsystem1 ==
  q : Inport
  Constant : Constant  Value=Lidar_2.pointing_b
  Constant1 : Constant  Value=Lidar_1.pointing_b
  Constant4 : Constant  Value=Lidar_2.Xb
  Constant5 : Constant  Value=Lidar_1.Xb
  Quaternion Rotation{,1..3} (4 alike) : aerolibutil/Quaternion Rotation
  vec_rot : Outport
  vec_rot1 : Outport  Port=2
  vec_rot2 : Outport  Port=3
  vec_rot3 : Outport  Port=4
  wires:
  q/1 -> Quaternion Rotation1/1, Quaternion Rotation/1, Quaternion Rotation3/1, Quaternion Rotation2/1
  Constant/1 -> Quaternion Rotation1/2
  Constant5/1 -> Quaternion Rotation2/2
  Quaternion Rotation2/1 -> vec_rot/1
  Constant4/1 -> Quaternion Rotation3/2
  Quaternion Rotation/1 -> vec_rot2/1
  Quaternion Rotation3/1 -> vec_rot1/1
  Constant1/1 -> Quaternion Rotation/2
  Quaternion Rotation1/1 -> vec_rot3/1

== matlab function FlightSim_6DOF/Sensors/IMU (VN-300)/Position ==
  data: pos_meas output; vel_meas output; pos_true input; vel_true input; dt input; sigma_pos input; sigma_vel input; tau_pos input; tau_vel input
function [pos_meas, vel_meas]= fcn(pos_true, vel_true, dt, sigma_pos, sigma_vel, tau_pos, tau_vel)
% pos = Inertial position ([m,m,m])
% vel = Inertial velocity ([m/s,m/s,m/s])
% dt = VN300 sample time (s)
% sigma_pos = steady-state standard deviation of position (RMS)
% sigma_vel = steady-state standard deviation of velocity (m/s)
% tau_pos = how long error persists (s)
% tau_vel = how long error persists (s)

persistent pos_error vel_error

if isempty(pos_error)
    pos_error = zeros(3,1);
    vel_error = zeros(3,1);
end

%% Time-Correlated Error
% GNSS measurements are time-correlated so errors can arise dependent on sample time
% This model is the first-order Gauss-Markov process
a_pos = exp(-dt/tau_pos);
a_vel = exp(-dt/tau_vel);

%% Total Error
pos_error = a_pos.*pos_error + sigma_pos.*sqrt(1-a_pos.^2).*randn(3,1);
vel_error = a_vel.*vel_error + sigma_vel.*sqrt(1-a_vel.^2).*randn(3,1);

pos_meas = pos_true + pos_error;
vel_meas = vel_true + vel_error;

== matlab function FlightSim_6DOF/Sensors/IMU (VN-300)/Attitude ==
  data: q_true input; q_meas_wb output; dt input; sigma_att input; tau_att input
function q_meas_wb = fcn(q_true, dt, sigma_att, tau_att)
% sigma_att = standard dev of [roll RMS, pitch RMS, heading RMS]
% tau_att = correlation time for attitude (s)

persistent att_error

if isempty(att_error)
    att_error = zeros(3,1);
end

%% Time Correlation 
% Like the position block, we'll use Guass-Markov Process

a = exp(-dt/tau_att);

att_error = a*att_error + sigma_att*sqrt(1-a^2).*randn(3,1);% [rads, rads, rads]

%% Quaternion error
q_error = [1;0.5*att_error]; % small angle approximation
q_error = q_error/norm(q_error); 

q_meas_wb = quatmultiply(q_true',q_error');
q_meas_wb = q_meas_wb/norm(q_meas_wb); % measured quaternion (earth to body)

== matlab function FlightSim_6DOF/Ranger Actuators/Commands to Required Moments ==
  data: roll_cmd input; pitch_cmd input; Mx_req output; yaw_cmd input; My_req output; I input; omega_b input; Mz_req output
function [Mx_req, My_req, Mz_req]= fcn(roll_cmd, pitch_cmd, yaw_cmd, I, omega_b)
    
    alpha_cmd = [roll_cmd; pitch_cmd; yaw_cmd];
    
    M_b_req = I*alpha_cmd + cross(omega_b, I*omega_b);
    
    Mx_req = M_b_req(1);   
    My_req = M_b_req(2);
    Mz_req = M_b_req(3);

== matlab function FlightSim_6DOF/Ranger Actuators/RCS ==
  data: Mx_req input; M_RCS output; I input
function M_RCS = fcn(Mx_req, I)
Ixx = I(1,1);

M_RCS = Mx_req;

== matlab function FlightSim_6DOF/Ranger Actuators/TVC ==
  data: My_req input; F_b output; Mz_req input; thrust_cmd input; L_engine input; M_b output; max_gimbal input
function [F_b, M_b] = fcn(My_req, Mz_req, thrust_cmd, L_engine, max_gimbal)
L = L_engine;
%% Eventually, we can add transient properties, that's why these are labeled as required/desired torques

dy_cmd = My_req / (thrust_cmd * L); % y-rotation gimbal angle from small angle approx
dz_cmd = Mz_req / (thrust_cmd * L); % z-rotation gimbal angle from small angle approx

dy_cmd = max(min(dy_cmd, max_gimbal), -max_gimbal); % limiting gimbal angles
dz_cmd = max(min(dz_cmd, max_gimbal), -max_gimbal);

u = [cos(dz_cmd)*cos(dy_cmd); sin(dz_cmd)*cos(dy_cmd); -sin(dy_cmd)];
F_b = thrust_cmd * u;
M_b = cross([-L;0;0], F_b);

%% The code above is temporary so that I can figure out some bugs

== matlab function FlightSim_6DOF/Hornet Actuators/Commands to Required Moments ==
  data: roll_cmd input; pitch_cmd input; Mx_req output; yaw_cmd input; My_req output; I input; omega_b input; Mz_req output
function [Mx_req, My_req, Mz_req]= fcn(roll_cmd, pitch_cmd, yaw_cmd, I, omega_b)
    
    alpha_cmd = [roll_cmd; pitch_cmd; yaw_cmd];
    
    M_b_req = I*alpha_cmd + cross(omega_b, I*omega_b);
    
    Mx_req = M_b_req(1);   
    My_req = M_b_req(2);
    Mz_req = M_b_req(3);

== matlab function FlightSim_6DOF/Hornet Actuators/RCS ==
  data: Mx_req input; M_RCS output; I input
function M_RCS = fcn(Mx_req, I)
Ixx = I(1,1);

M_RCS = Mx_req;

== matlab function FlightSim_6DOF/Flight Controller/MATLAB Function ==
  data: world_tilt_x input; z_des_w output; world_tilt_y input; max_tilt_rad input
function z_des_w = fcn(world_tilt_x, world_tilt_y, max_tilt_rad)

world_tilt_x = clip(world_tilt_x, -max_tilt_rad, max_tilt_rad);
world_tilt_y = clip(world_tilt_y, -max_tilt_rad, max_tilt_rad);

z = [tan(world_tilt_x); tan(world_tilt_y); 1];
z_des_w = z / norm(z);

end

== matlab function FlightSim_6DOF/Hornet Actuators/TVC ==
  data: My_req input; F_b output; Mz_req input; thrust_cmd input; L_engine input; M_b output; max_gimbal input
function [F_b, M_b] = fcn(My_req, Mz_req, thrust_cmd, L_engine, max_gimbal)
L = L_engine;
%% Eventually, we can add transient properties, that's why these are labeled as required/desired torques

dy_cmd = My_req / (thrust_cmd * L); % y-rotation gimbal angle from small angle approx
dz_cmd = Mz_req / (thrust_cmd * L); % z-rotation gimbal angle from small angle approx

dy_cmd = max(min(dy_cmd, max_gimbal), -max_gimbal); % limiting gimbal angles
dz_cmd = max(min(dz_cmd, max_gimbal), -max_gimbal);

u = [cos(dz_cmd)*cos(dy_cmd); sin(dz_cmd)*cos(dy_cmd); -sin(dy_cmd)];
F_b = thrust_cmd * u;
M_b = cross([-L;0;0], F_b);

%% The code above is temporary so that I can figure out some bugs

== matlab function FlightSim_6DOF/Ground Contact ==
  data: X_e input; V_e input; F_b output; DCM_be input; M_b output; w_b input; Fn output; inContact output; g parameter; veh parameter; feet_pos_body_m parameter
function [F_b, M_b, Fn, inContact] = groundContact(X_e, V_e, DCM_be, w_b, g, veh, feet_pos_body_m)
m = veh.m; % vehicle mass from FS_6DOF_config.m
% Based on "A Fast and Stable Penalty Method for Rigid Body Simulation"
% https://ieeexplore.ieee.org/document/4359964

up_earth = [1; 0; 0];
k = m*g/(4*0.01);
c = 2*0.7*sqrt(k*m/4);

x = X_e(:);
C_eb = DCM_be.';

F_b = zeros(3,1);
M_b = zeros(3,1);
Fn = zeros(4,1);
inContact = zeros(4,1);

for i = 1:4
    ri = feet_pos_body_m(:,i);
    foot_pos_earth = x + C_eb*ri;
    h = up_earth.'*foot_pos_earth;

    if h < 0
        pen = -h;
        v_foot = V_e(:) + C_eb*cross(w_b(:), ri);
        vn    = up_earth.'*v_foot;
        fn    = max(k*pen - c*vn, 0);
        f_e = fn*up_earth;
        f_b = DCM_be*f_e;

        F_b = F_b + f_b;
        M_b = M_b + cross(ri, f_b);
        Fn(i) = fn;
        inContact(i) = 1;
    end
end
end

== matlab function FlightSim_6DOF/Sensors/Lidar #1 and #2 (TF02-Pro)1 ==
  data: lidar1_offset_w input; lidar2_offset_w input; range_meas1 output; range_meas2 output; pointing1_w input; pointing2_w input; max_range input; lidar_std input; Xe input
function [range_meas1, range_meas2]= fcn(lidar1_offset_w, lidar2_offset_w, pointing1_w, pointing2_w, max_range, lidar_std, Xe)
% lidar_offset_w = lidar offset from Xe, [x_w, y_w, z_w]
% pointing = inertial lidar pointing vector
% max_range = maximum rangefinder depth, m
% lidar_std = standard deviation of lidar data
% Xe = vehicle CG position in world frame


% ground is flat and at inertial z = 0 m
z_ground = 0;

% add sensor cg offset to cg position to get world position
lidar1_pos_w = lidar1_offset_w + Xe;
lidar2_pos_w = lidar2_offset_w + Xe;

% normalize
pointing1_w_unit = pointing1_w/norm(pointing1_w);
pointing2_w_unit = pointing2_w/norm(pointing2_w);

% angle to horizontal = angle to ground
ang1 = (pointing1_w_unit(3)); % sine of angle b/w lidar pointing and horizontal
ang2 = (pointing2_w_unit(3));


%% lidar 1
if abs(sin(ang1)) < 1e-6
    % Beam is parallel to the ground -- never intersects
    range_meas1 = max_range;
else
    t = (z_ground+lidar1_pos_w(3))/ang1;
    if t <= 0 || t > max_range
        % Ground is behind the beam, or intersection is beyond sensor range
        range_meas1 = max_range;      % or NaN, depending on how your estimator handles no-return
    else
        noise = randn(1)*(lidar_std);
        range_meas1 = t +  noise;
    end
end

%% lidar 2
if abs(sin(ang2)) < 1e-6
    % Beam is parallel to the ground -- never intersects
    range_meas2 = max_range;
else
    t = (z_ground+lidar2_pos_w(3))/ang2;
    if t <= 0 || t > max_range
        % Ground is behind the beam, or intersection is beyond sensor range
        range_meas2 = max_range;      % or NaN, depending on how your estimator handles no-return
    else
        noise = randn(1)*(lidar_std);
        range_meas2 = t +  noise;
    end
end
